simulink model "EV_Truck_Model"  (R2022b)
settings: Solver=FixedStepAuto  StartTime=0  StopTime=26553  FixedStep=0.1  RelTol=1e-3
model workspace (MAT data in the model file):
  ADAS_MaxAccel = 2
  ADAS_MaxDecel = 2.5
  Adas_on_off = 0
  Batt_cap_ah : Simulink.Parameter (value not decoded)
  Batt_rist_r0 : Simulink.Parameter (value not decoded)
  Batt_soc_s0 : Simulink.Parameter (value not decoded)
  Batt_volt_v0 : Simulink.Parameter (value not decoded)
  Motor_eff_100 : Simulink.Parameter (value not decoded)
  Motor_eff_190 : Simulink.Parameter (value not decoded)
  Motor_eff_95 : Simulink.Parameter (value not decoded)
  Motor_rpm_100 : Simulink.Parameter (value not decoded)
  Motor_rpm_190 : Simulink.Parameter (value not decoded)
  Motor_rpm_95 : Simulink.Parameter (value not decoded)
  Motor_torque_pos_100 : Simulink.Parameter (value not decoded)
  Motor_torque_pos_190 : Simulink.Parameter (value not decoded)
  Motor_torque_pos_95 : Simulink.Parameter (value not decoded)
  Motor_trq_190 : Simulink.Parameter (value not decoded)
  Motor_trq_95 : Simulink.Parameter (value not decoded)
  Sim_step = 0.1
  Test_DriveCycle = 0
  Trans_ratio = 6.142
  Veh_cog_fx = 1.69543
  Veh_cog_h = 0.605887
  Veh_cog_rx = 2.11956
  Veh_diff = 6.7
  Veh_whl_crr = 0.01
  Veh_whl_k = 180000
  Veh_whl_radius = 0.35
symbols that are objects in the model workspace (value not decoded): Motor_eff_100, Motor_eff_190, Motor_eff_95, Motor_rpm_100, Motor_rpm_190, Motor_rpm_95, Motor_torque_pos_100, Motor_torque_pos_190, Motor_torque_pos_95, Motor_trq_190, Motor_trq_95
undefined symbols (not defined in the file): Batt_soc_init, canChannel, Elec_aux_sw, Elec_rgn_sw, Power_option, speed, time, Veh_mass
libraries: batteryecm_lib x170, simulink x14, canmsglib x9, canlib x7, autolibshared x5, nesl_utility x4, fl_lib x3, drivingvehiclecontroller x3, hdlsllib x3, sim3dlib x1, sim3dautolib x1, vrlib x1
(part 11 of 11)

== stateflow chart EV_Truck_Model/VCU/Remap Subsystem/VCU_TorqueCommand ==
  state CruiseControl [commented out]
    state TooSlow [commented out]
      TrqCmd = TrqCmd + 5* ...
      abs(Speed-ADAS_speed);
      state NoBrake [commented out]
      state Brake [commented out]
        BrakeCmd = ...
        BrakeCmd + 5;
      (default) -> NoBrake [commented out]
      NoBrake -> CruiseControl.TooSlow.Brake [commented out] : [TrqCmd<0]
    state InitialState [commented out]
      TrqCmd = 100;
    state TooFast [commented out]
      TrqCmd = TrqCmd - 5* ...
      abs(Speed-ADAS_speed);
      BrakeCmd = 0;
    state PerfectCondition [commented out]
      %No Command
    state Error [commented out]
      ADAS_fault = 1;
    state TempState [commented out]
      %Wait 0.1 sec
    (default) -> InitialState [commented out]
    InitialState -> PerfectCondition [commented out]
    (junction 250) -> TooFast [commented out] : [Speed > ADAS_speed+2.0]
    (junction 250) -> TooSlow [commented out] : [Speed < ADAS_speed-2.0]
    (junction 250) -> Error [commented out] : [abs(Speed-ADAS_speed)>10]
    TooFast -> TempState [commented out]
    PerfectCondition -> (junction 250) [commented out]
    TempState -> PerfectCondition [commented out] : after(0.1,sec)
    TooSlow -> TempState [commented out]
  state AdaptiveCruiseControl [commented out]
    TargetDistance = Speed*(1+(ADAS_mode-3)*0.1)/2+1;
    if 1/TTC < 0.1
    ADAS_SpdCmd = ADAS_speed;
    else
    ADAS_SpdCmd = ADAS_speed;
    end
  state Initialize
    state BOTS [parallel]
      settings: executionOrder=1
      state BrakeFactor0
        BrakeFactor=0;
      state BrakeFactor1
        BrakeFactor=1;
      Initialize.BOTS.BrakeFactor0 -> Initialize.BOTS.BrakeFactor1 : [Brake > 0]
      (default) -> Initialize.BOTS.BrakeFactor1
      Initialize.BOTS.BrakeFactor1 -> Initialize.BOTS.BrakeFactor0 : [Brake == 0]
    state RegenTriggerCriteria [parallel]
      settings: executionOrder=2
      state RegenOff
        Regen = 0;
        DCRegen = 0;
      state RegenOn
        Regen = 1;
        DCRegen = 1;
      RegenOff -> RegenOn : [RPM>200&&(RegenSW==1||DCRegenSW==1)&&SOC<=0.95]
      (default) -> RegenOff
      RegenOn -> RegenOff : [RPM<200||(RegenSW==0&&DCRegenSW==0)||SOC>0.95]
    state DriveCycleTset [parallel] [commented out]
    state ADASTriggerCriteria [parallel]
      settings: executionOrder=3
      state CruiseOff
        ADAS = 0;
        ADAS_fault = 0;
      state CruiseOn
        ADAS = 1;
        state PLUSTEMP
          %Stop increase
        state PLUS
          ADAS_speed...
          =ADAS_speed+1;
        state PLUSTEMP5
          %Stop increase
        state PLUS5
          ADAS_speed...
          =ADAS_speed+5;
        state IC
          ADAS_speed = ...
          Speed;
          %1 Time Only
        state NC
          %No Command
        state MINUSTEMP
          %Stop decrease
        state MINUS
          ADAS_speed...
          =ADAS_speed-1;
        state MINUSTEMP5
          %Stop decrease
        state MINUS5
          ADAS_speed...
          =ADAS_speed-5;
        PLUSTEMP -> PLUS5 [order 2] : after(0.75,sec)
        PLUS5 -> PLUSTEMP5
        NC -> PLUSTEMP [order 1] : [ADAS_add == 1]
        PLUSTEMP5 -> (junction 376) [order 2] : [ADAS_add == 0]
        PLUS -> (junction 215)
        PLUSTEMP -> PLUS [order 1] : [ADAS_add == 0]
        PLUSTEMP5 -> PLUS5 [order 1] : after(0.25,sec)
        (default) -> IC
        (junction 376) -> (junction 215)
        (junction 215) -> NC
        MINUSTEMP5 -> (junction 376) [order 2] : [ADAS_min == 0]
        MINUS -> (junction 215)
        IC -> NC
        MINUS5 -> MINUSTEMP5
        MINUSTEMP -> MINUS [order 2] : [ADAS_min == 0]
        NC -> MINUSTEMP [order 2] : [ADAS_min == 1]
        MINUSTEMP -> MINUS5 [order 1] : after(0.75,sec)
        MINUSTEMP5 -> MINUS5 [order 1] : after(0.25,sec)
      state CruiseReady
        ADAS = 0;
        ADAS_speed ...
        =0;
      state CruiseTest
        ADAS = 1;
        ADAS_speed=ADAS_speed_profile;
      CruiseReady -> CruiseOff [order 2] : [ADAS_on == 0]
      (default) -> CruiseOff
      CruiseOn -> CruiseReady : [ADAS_enable == 0 || ADAS_on == 0 || ADAS_fault == 1 || BrakeFactor ==1]
      CruiseOff -> CruiseReady : [ADAS_on == 1]
      CruiseReady -> CruiseTest [order 3] : [ADAS_test == 1]
      CruiseReady -> CruiseOn [order 1] : [ADAS_enable == 1 && BrakeFactor== 0 && Speed > 20]
    state ThrottleMapping [parallel]
      settings: executionOrder=4
      state Initiation
        ADAS_SpdCmd = 0;
        state CruiseControl
          state TrqCmdMapping [parallel]
            settings: executionOrder=1
            state NoRegen
              TrqCmd = ADAS_AccelCmd ...
              /2*600;
              BrakeCmd = ADAS_DecelCmd ...
              /2.5*600;
            state Regen
              TrqCmd = ADAS_AccelCmd ...
              /2*600;
              BrakeCmd = ADAS_DecelCmd ...
              /2.5*600;
            state AdaptiveCruiseControlException
              TrqCmd = 0;
            Regen -> NoRegen [order 1] : [Regen == 0]
            NoRegen -> Regen [order 1] : [Regen == 1]
            NoRegen -> (junction 412) [order 2]
            Regen -> (junction 412) [order 2]
            (junction 412) -> AdaptiveCruiseControlException : [ADAS_exception == 1]
            AdaptiveCruiseControlException -> NoRegen : [ADAS_exception == 0]
          state ControlState [parallel]
            ADAS_activate = 1;
            settings: executionOrder=2
            state CruiseControl
              ADAS_SpdCmd = ADAS_speed;
              state ErrorState
                ADAS_fault = 1;
                ADAS_activate = 0;
              state ErrorCheck
              ErrorCheck -> ErrorState : [abs(Speed-ADAS_speed)>10 && after(1,sec)&&ADAS_test==0]
              (default) -> ErrorCheck
            state AdaptiveCruiseControl
              TargetDistance = Speed* ...
              (1+(ADAS_mode-3)*0.1)/2+0.5;
              if ADAS_SpdCmd > ADAS_speed
              ADAS_SpdCmd = ADAS_speed;
              end
              state Brake
                ADAS_exception =1;
                ADAS_SpdCmd = 5;
                state CrashDanger
                  BrakeCmd = 1000;
                state ApplyBrake
                  BrakeCmd = 500/TTC;
                ApplyBrake -> CrashDanger : [TTC<0.5]
                CrashDanger -> ApplyBrake : [TTC>=0.5]
                (default) -> ApplyBrake
              state StillFarAway
                ADAS_SpdCmd = ADAS_speed;
                if ADAS_Speed_Deltakph < -10
                ADAS_SpdCmd = Speed+ ...
                ADAS_Speed_Deltakph/ ...
                (ADAS_Distance- ...
                TargetDistance);
                elseif ADAS_Speed_Deltakph > 5
                ADAS_SpdCmd = Speed+ ...
                ADAS_Speed_Deltakph;
                end
                if ADAS_SpdCmd > ADAS_speed
                ADAS_SpdCmd = ADAS_speed;
                end
              state TooFarAway
                ADAS_SpdCmd ...
                = ADAS_speed;
              state MaintainDistance
                ADAS_SpdCmd = Speed+ ...
                ADAS_Speed_Deltakph;
                ADAS_exception =0;
                if ADAS_SpdCmd > ADAS_speed
                ADAS_SpdCmd = ADAS_speed;
                end
              Initialize.ThrottleMapping.Initiation.CruiseControl.ControlState.AdaptiveCruiseControl.Brake -> MaintainDistance : [TTC>=5]
              MaintainDistance -> Initialize.ThrottleMapping.Initiation.CruiseControl.ControlState.AdaptiveCruiseControl.Brake [order 2] : [TTC<5]
              (default) -> TooFarAway
              StillFarAway -> TooFarAway [order 2] : [ADAS_Distance >= 200]
              TooFarAway -> StillFarAway : [ADAS_Distance < 200]
              MaintainDistance -> StillFarAway [order 1] : [ADAS_Distance >= TargetDistance]
              StillFarAway -> MaintainDistance [order 1] : [ADAS_Distance < TargetDistance]
            (default) -> Initialize.ThrottleMapping.Initiation.CruiseControl.ControlState.CruiseControl
            Initialize.ThrottleMapping.Initiation.CruiseControl.ControlState.CruiseControl -> Initialize.ThrottleMapping.Initiation.CruiseControl.ControlState.AdaptiveCruiseControl : [ADAS_mode ~= 0]
            Initialize.ThrottleMapping.Initiation.CruiseControl.ControlState.AdaptiveCruiseControl -> Initialize.ThrottleMapping.Initiation.CruiseControl.ControlState.CruiseControl : [ADAS_mode == 0]
          (default) -> NoRegen
        state ForwardGear
          ADAS_activate = 0;
          state OPD
            state TrqCmd_Regen
              state TrqCmd_Positive
                TrqCmd = TrqLimit_Pos* ...
                (Throttle-40)/160;
                BrakeCmd = 0;
              state TrqCmd_Negative
                TrqCmd = ...
                -100+100 ...
                *Throttle/40;
                BrakeCmd = 0;
              state Brake
                state Brake_RGN
                  TrqCmd = -100 ...
                  -200*Brake/150;
                  BrakeCmd = 450 ...
                  *Brake/150;
                state Brake_NoTrq
                  TrqCmd = 0;
                  BrakeCmd = ...
                  Brake*5;
                (default) -> Initialize.ThrottleMapping.Initiation.ForwardGear.OPD.TrqCmd_Regen.Brake.Brake_RGN
                Initialize.ThrottleMapping.Initiation.ForwardGear.OPD.TrqCmd_Regen.Brake.Brake_NoTrq -> Initialize.ThrottleMapping.Initiation.ForwardGear.OPD.TrqCmd_Regen.Brake.Brake_RGN : [Brake < 150]
                Initialize.ThrottleMapping.Initiation.ForwardGear.OPD.TrqCmd_Regen.Brake.Brake_RGN -> Initialize.ThrottleMapping.Initiation.ForwardGear.OPD.TrqCmd_Regen.Brake.Brake_NoTrq : [Brake > 150]
              (default) -> Initialize.ThrottleMapping.Initiation.ForwardGear.OPD.TrqCmd_Regen.TrqCmd_Positive
              Initialize.ThrottleMapping.Initiation.ForwardGear.OPD.TrqCmd_Regen.TrqCmd_Negative -> Initialize.ThrottleMapping.Initiation.ForwardGear.OPD.TrqCmd_Regen.TrqCmd_Positive [order 2] : [Throttle >= 40]
              Initialize.ThrottleMapping.Initiation.ForwardGear.OPD.TrqCmd_Regen.TrqCmd_Positive -> Initialize.ThrottleMapping.Initiation.ForwardGear.OPD.TrqCmd_Regen.TrqCmd_Negative [order 1] : [Throttle < 40]
              Initialize.ThrottleMapping.Initiation.ForwardGear.OPD.TrqCmd_Regen.TrqCmd_Positive -> (junction 74) [order 2]
              Initialize.ThrottleMapping.Initiation.ForwardGear.OPD.TrqCmd_Regen.TrqCmd_Negative -> (junction 74) [order 1]
              (junction 74) -> Initialize.ThrottleMapping.Initiation.ForwardGear.OPD.TrqCmd_Regen.Brake : [BrakeFactor ==1]
              Initialize.ThrottleMapping.Initiation.ForwardGear.OPD.TrqCmd_Regen.Brake -> Initialize.ThrottleMapping.Initiation.ForwardGear.OPD.TrqCmd_Regen.TrqCmd_Negative : [BrakeFactor == 0]
            state NoTrqCmd
              TrqCmd = 0;
              BrakeCmd = ...
              Brake*5;
            state TrqCmd_Normal
              TrqCmd = ...
              TrqLimit_Pos*...
              Throttle/200;
              BrakeCmd = 0;
            (default) -> Initialize.ThrottleMapping.Initiation.ForwardGear.OPD.NoTrqCmd
            Initialize.ThrottleMapping.Initiation.ForwardGear.OPD.TrqCmd_Normal -> Initialize.ThrottleMapping.Initiation.ForwardGear.OPD.NoTrqCmd [order 2] : [BrakeFactor == 1]
            Initialize.ThrottleMapping.Initiation.ForwardGear.OPD.NoTrqCmd -> Initialize.ThrottleMapping.Initiation.ForwardGear.OPD.TrqCmd_Normal : [BrakeFactor == 0]
            Initialize.ThrottleMapping.Initiation.ForwardGear.OPD.TrqCmd_Regen -> Initialize.ThrottleMapping.Initiation.ForwardGear.OPD.TrqCmd_Normal : [Regen == 0]
            Initialize.ThrottleMapping.Initiation.ForwardGear.OPD.TrqCmd_Normal -> Initialize.ThrottleMapping.Initiation.ForwardGear.OPD.TrqCmd_Regen [order 1] : [Regen == 1]
          state non_OPD
            state TrqCmd_Regen
              state TrqCmd
                TrqCmd = TrqLimit_Pos* ...
                Throttle/200;
                BrakeCmd = 0;
              state Brake
                state Brake_RGN
                  TrqCmd = -300* ...
                  Brake/150;
                  BrakeCmd = 450 ...
                  *Brake/150;
                state Brake_NoTrq
                  TrqCmd = 0;
                  BrakeCmd = ...
                  Brake*5;
                (default) -> Initialize.ThrottleMapping.Initiation.ForwardGear.non_OPD.TrqCmd_Regen.Brake.Brake_RGN
                Initialize.ThrottleMapping.Initiation.ForwardGear.non_OPD.TrqCmd_Regen.Brake.Brake_NoTrq -> Initialize.ThrottleMapping.Initiation.ForwardGear.non_OPD.TrqCmd_Regen.Brake.Brake_RGN : [Brake < 150]
                Initialize.ThrottleMapping.Initiation.ForwardGear.non_OPD.TrqCmd_Regen.Brake.Brake_RGN -> Initialize.ThrottleMapping.Initiation.ForwardGear.non_OPD.TrqCmd_Regen.Brake.Brake_NoTrq : [Brake > 150]
              (default) -> Initialize.ThrottleMapping.Initiation.ForwardGear.non_OPD.TrqCmd_Regen.TrqCmd
              Initialize.ThrottleMapping.Initiation.ForwardGear.non_OPD.TrqCmd_Regen.Brake -> Initialize.ThrottleMapping.Initiation.ForwardGear.non_OPD.TrqCmd_Regen.TrqCmd : [BrakeFactor == 0]
              Initialize.ThrottleMapping.Initiation.ForwardGear.non_OPD.TrqCmd_Regen.TrqCmd -> Initialize.ThrottleMapping.Initiation.ForwardGear.non_OPD.TrqCmd_Regen.Brake : [BrakeFactor == 1]
            state NoTrqCmd
              TrqCmd = 0;
              BrakeCmd = ...
              Brake*5;
            state TrqCmd_Normal
              TrqCmd = ...
              TrqLimit_Pos*...
              Throttle/200;
              BrakeCmd = 0;
            (default) -> Initialize.ThrottleMapping.Initiation.ForwardGear.non_OPD.NoTrqCmd
            Initialize.ThrottleMapping.Initiation.ForwardGear.non_OPD.TrqCmd_Normal -> Initialize.ThrottleMapping.Initiation.ForwardGear.non_OPD.NoTrqCmd [order 2] : [BrakeFactor == 1]
            Initialize.ThrottleMapping.Initiation.ForwardGear.non_OPD.NoTrqCmd -> Initialize.ThrottleMapping.Initiation.ForwardGear.non_OPD.TrqCmd_Normal : [BrakeFactor == 0]
            Initialize.ThrottleMapping.Initiation.ForwardGear.non_OPD.TrqCmd_Regen -> Initialize.ThrottleMapping.Initiation.ForwardGear.non_OPD.TrqCmd_Normal : [Regen == 0]
            Initialize.ThrottleMapping.Initiation.ForwardGear.non_OPD.TrqCmd_Normal -> Initialize.ThrottleMapping.Initiation.ForwardGear.non_OPD.TrqCmd_Regen [order 1] : [Regen == 1]
          Initialize.ThrottleMapping.Initiation.ForwardGear.OPD -> Initialize.ThrottleMapping.Initiation.ForwardGear.non_OPD : [OPDSW == 0]
          Initialize.ThrottleMapping.Initiation.ForwardGear.non_OPD -> Initialize.ThrottleMapping.Initiation.ForwardGear.OPD : [OPDSW == 1]
          (default) -> Initialize.ThrottleMapping.Initiation.ForwardGear.non_OPD
        state NeutralGear
          TrqCmd = 0;
          BrakeCmd = Brake*5;
        state ReverseGear
          TrqCmd = Throttle/200* ...
          TrqLimit_Neg*0.75;
          BrakeCmd = Brake*5;
        (default) -> Initialize.ThrottleMapping.Initiation.NeutralGear
        (junction 319) -> Initialize.ThrottleMapping.Initiation.NeutralGear : [Gear == 0]
        Initialize.ThrottleMapping.Initiation.NeutralGear -> (junction 317) [order 2]
        Initialize.ThrottleMapping.Initiation.NeutralGear -> (junction 315) [order 1]
        Initialize.ThrottleMapping.Initiation.ForwardGear -> (junction 319) [order 2]
        Initialize.ThrottleMapping.Initiation.ReverseGear -> (junction 319) [order 2]
        (junction 315) -> Initialize.ThrottleMapping.Initiation.ForwardGear : [Gear ==1]
        Initialize.ThrottleMapping.Initiation.ReverseGear -> (junction 315) [order 1]
        Initialize.ThrottleMapping.Initiation.ForwardGear -> (junction 317) [order 3]
        (junction 317) -> Initialize.ThrottleMapping.Initiation.ReverseGear : [Gear == 2]
        Initialize.ThrottleMapping.Initiation.ForwardGear -> Initialize.ThrottleMapping.Initiation.CruiseControl [order 1] : [ADAS == 1]
        Initialize.ThrottleMapping.Initiation.CruiseControl -> Initialize.ThrottleMapping.Initiation.ForwardGear : [ADAS == 0]
      state DriveCycleTest
        ADAS_SpdCmd = 0;
        note: Throttle Command 0-200
            | Brake Command 0-200
            | 4 State:
            | OPD on/off
            | RGN on/off
        state TorqueCommand [parallel]
          settings: executionOrder=1
          state ForwardGear
            ADAS_activate = 0;
            state OPD [commented out]
              state TrqCmd_Regen [commented out]
                state TrqCmd_Positive [commented out]
                  TrqCmd = TrqLimit_Pos* ...
                  (DCThrottle-40)/160;
                  BrakeCmd = 0;
                state TrqCmd_Negative [commented out]
                  TrqCmd = ...
                  -100+100 ...
                  *DCThrottle/40;
                  BrakeCmd = 0;
                state Brake [commented out]
                  state Brake_RGN [commented out]
                    TrqCmd = -100 ...
                    -200*DCBrake/150;
                    BrakeCmd = 450 ...
                    *DCBrake/150;
                  state Brake_NoTrq [commented out]
                    TrqCmd = 0;
                    BrakeCmd = ...
                    DCBrake*5;
                  (default) -> Initialize.ThrottleMapping.DriveCycleTest.TorqueCommand.ForwardGear.OPD.TrqCmd_Regen.Brake.Brake_RGN [commented out]
                  Initialize.ThrottleMapping.DriveCycleTest.TorqueCommand.ForwardGear.OPD.TrqCmd_Regen.Brake.Brake_NoTrq -> Initialize.ThrottleMapping.DriveCycleTest.TorqueCommand.ForwardGear.OPD.TrqCmd_Regen.Brake.Brake_RGN [commented out] : [DCBrake < 150]
                  Initialize.ThrottleMapping.DriveCycleTest.TorqueCommand.ForwardGear.OPD.TrqCmd_Regen.Brake.Brake_RGN -> Initialize.ThrottleMapping.DriveCycleTest.TorqueCommand.ForwardGear.OPD.TrqCmd_Regen.Brake.Brake_NoTrq [commented out] : [DCBrake > 150]
                (default) -> Initialize.ThrottleMapping.DriveCycleTest.TorqueCommand.ForwardGear.OPD.TrqCmd_Regen.TrqCmd_Positive [commented out]
                Initialize.ThrottleMapping.DriveCycleTest.TorqueCommand.ForwardGear.OPD.TrqCmd_Regen.TrqCmd_Negative -> Initialize.ThrottleMapping.DriveCycleTest.TorqueCommand.ForwardGear.OPD.TrqCmd_Regen.TrqCmd_Positive [commented out] : [DCThrottle >= 40]
                Initialize.ThrottleMapping.DriveCycleTest.TorqueCommand.ForwardGear.OPD.TrqCmd_Regen.TrqCmd_Positive -> Initialize.ThrottleMapping.DriveCycleTest.TorqueCommand.ForwardGear.OPD.TrqCmd_Regen.TrqCmd_Negative [commented out] : [DCThrottle < 40]
                Initialize.ThrottleMapping.DriveCycleTest.TorqueCommand.ForwardGear.OPD.TrqCmd_Regen.TrqCmd_Positive -> (junction 435) [commented out]
                Initialize.ThrottleMapping.DriveCycleTest.TorqueCommand.ForwardGear.OPD.TrqCmd_Regen.TrqCmd_Negative -> (junction 435) [commented out]
                (junction 435) -> Initialize.ThrottleMapping.DriveCycleTest.TorqueCommand.ForwardGear.OPD.TrqCmd_Regen.Brake [commented out] : [DCBrakeFactor ==1]
                Initialize.ThrottleMapping.DriveCycleTest.TorqueCommand.ForwardGear.OPD.TrqCmd_Regen.Brake -> Initialize.ThrottleMapping.DriveCycleTest.TorqueCommand.ForwardGear.OPD.TrqCmd_Regen.TrqCmd_Negative [commented out] : [DCBrakeFactor == 0]
              state NoTrqCmd [commented out]
                TrqCmd = 0;
                BrakeCmd = ...
                DCBrake*5;
              state TrqCmd_Normal [commented out]
                TrqCmd = ...
                TrqLimit_Pos*...
                DCThrottle/200;
                BrakeCmd = 0;
              (default) -> Initialize.ThrottleMapping.DriveCycleTest.TorqueCommand.ForwardGear.OPD.NoTrqCmd [commented out]
              Initialize.ThrottleMapping.DriveCycleTest.TorqueCommand.ForwardGear.OPD.TrqCmd_Normal -> Initialize.ThrottleMapping.DriveCycleTest.TorqueCommand.ForwardGear.OPD.NoTrqCmd [commented out] : [BrakeFactor == 1]
              Initialize.ThrottleMapping.DriveCycleTest.TorqueCommand.ForwardGear.OPD.NoTrqCmd -> Initialize.ThrottleMapping.DriveCycleTest.TorqueCommand.ForwardGear.OPD.TrqCmd_Normal [commented out] : [BrakeFactor == 0]
              Initialize.ThrottleMapping.DriveCycleTest.TorqueCommand.ForwardGear.OPD.TrqCmd_Regen -> Initialize.ThrottleMapping.DriveCycleTest.TorqueCommand.ForwardGear.OPD.TrqCmd_Normal [commented out] : [Regen == 0]
              Initialize.ThrottleMapping.DriveCycleTest.TorqueCommand.ForwardGear.OPD.TrqCmd_Normal -> Initialize.ThrottleMapping.DriveCycleTest.TorqueCommand.ForwardGear.OPD.TrqCmd_Regen [commented out] : [Regen == 1]
            state non_OPD
              state TrqCmd_Regen
                state TrqCmd
                  TrqCmd = TrqLimit_Pos* ...
                  DCThrottle/200;
                  BrakeCmd = 0;
                state Brake
                  state Brake_RGN
                    TrqCmd = -300* ...
                    DCBrake/150;
                    BrakeCmd = 450 ...
                    *DCBrake/150;
                  state Brake_NoTrq
                    TrqCmd = 0;
                    BrakeCmd = ...
                    DCBrake*5;
                  (default) -> Initialize.ThrottleMapping.DriveCycleTest.TorqueCommand.ForwardGear.non_OPD.TrqCmd_Regen.Brake.Brake_RGN
                  Initialize.ThrottleMapping.DriveCycleTest.TorqueCommand.ForwardGear.non_OPD.TrqCmd_Regen.Brake.Brake_NoTrq -> Initialize.ThrottleMapping.DriveCycleTest.TorqueCommand.ForwardGear.non_OPD.TrqCmd_Regen.Brake.Brake_RGN : [DCBrake < 150]
                  Initialize.ThrottleMapping.DriveCycleTest.TorqueCommand.ForwardGear.non_OPD.TrqCmd_Regen.Brake.Brake_RGN -> Initialize.ThrottleMapping.DriveCycleTest.TorqueCommand.ForwardGear.non_OPD.TrqCmd_Regen.Brake.Brake_NoTrq : [DCBrake > 150]
                (default) -> Initialize.ThrottleMapping.DriveCycleTest.TorqueCommand.ForwardGear.non_OPD.TrqCmd_Regen.TrqCmd
                Initialize.ThrottleMapping.DriveCycleTest.TorqueCommand.ForwardGear.non_OPD.TrqCmd_Regen.Brake -> Initialize.ThrottleMapping.DriveCycleTest.TorqueCommand.ForwardGear.non_OPD.TrqCmd_Regen.TrqCmd : [DCBrakeFactor == 0]
                Initialize.ThrottleMapping.DriveCycleTest.TorqueCommand.ForwardGear.non_OPD.TrqCmd_Regen.TrqCmd -> Initialize.ThrottleMapping.DriveCycleTest.TorqueCommand.ForwardGear.non_OPD.TrqCmd_Regen.Brake : [DCBrakeFactor == 1]
              state NoTrqCmd
                TrqCmd = 0;
                BrakeCmd = ...
                DCBrake*5;
              state TrqCmd_Normal
                TrqCmd = ...
                TrqLimit_Pos*...
                DCThrottle/200;
                BrakeCmd = 0;
              (default) -> Initialize.ThrottleMapping.DriveCycleTest.TorqueCommand.ForwardGear.non_OPD.NoTrqCmd
              Initialize.ThrottleMapping.DriveCycleTest.TorqueCommand.ForwardGear.non_OPD.TrqCmd_Normal -> Initialize.ThrottleMapping.DriveCycleTest.TorqueCommand.ForwardGear.non_OPD.NoTrqCmd [order 1] : [DCBrakeFactor == 1]
              Initialize.ThrottleMapping.DriveCycleTest.TorqueCommand.ForwardGear.non_OPD.NoTrqCmd -> Initialize.ThrottleMapping.DriveCycleTest.TorqueCommand.ForwardGear.non_OPD.TrqCmd_Normal : [DCBrakeFactor == 0]
              Initialize.ThrottleMapping.DriveCycleTest.TorqueCommand.ForwardGear.non_OPD.TrqCmd_Regen -> Initialize.ThrottleMapping.DriveCycleTest.TorqueCommand.ForwardGear.non_OPD.TrqCmd_Normal : [DCRegen == 0]
              Initialize.ThrottleMapping.DriveCycleTest.TorqueCommand.ForwardGear.non_OPD.TrqCmd_Normal -> Initialize.ThrottleMapping.DriveCycleTest.TorqueCommand.ForwardGear.non_OPD.TrqCmd_Regen [order 2] : [DCRegen == 1]
            Initialize.ThrottleMapping.DriveCycleTest.TorqueCommand.ForwardGear.OPD -> Initialize.ThrottleMapping.DriveCycleTest.TorqueCommand.ForwardGear.non_OPD [commented out] : [OPDSW == 0]
            Initialize.ThrottleMapping.DriveCycleTest.TorqueCommand.ForwardGear.non_OPD -> Initialize.ThrottleMapping.DriveCycleTest.TorqueCommand.ForwardGear.OPD [commented out] : [OPDSW == 1]
            (default) -> Initialize.ThrottleMapping.DriveCycleTest.TorqueCommand.ForwardGear.non_OPD
          state NeutralGear
            TrqCmd = 0;
            BrakeCmd = DCBrake*5;
          state ReverseGear
            TrqCmd = DCThrottle/200* ...
            TrqLimit_Neg*0.75;
            BrakeCmd = DCBrake*5;
          (default) -> Initialize.ThrottleMapping.DriveCycleTest.TorqueCommand.NeutralGear
          (junction 488) -> Initialize.ThrottleMapping.DriveCycleTest.TorqueCommand.NeutralGear : [Gear == 0]
          Initialize.ThrottleMapping.DriveCycleTest.TorqueCommand.NeutralGear -> (junction 463) [order 2]
          Initialize.ThrottleMapping.DriveCycleTest.TorqueCommand.NeutralGear -> (junction 471) [order 1]
          Initialize.ThrottleMapping.DriveCycleTest.TorqueCommand.ForwardGear -> (junction 488) [order 1]
          Initialize.ThrottleMapping.DriveCycleTest.TorqueCommand.ReverseGear -> (junction 488) [order 2]
          (junction 471) -> Initialize.ThrottleMapping.DriveCycleTest.TorqueCommand.ForwardGear : [Gear ==1]
          Initialize.ThrottleMapping.DriveCycleTest.TorqueCommand.ReverseGear -> (junction 471) [order 1]
          Initialize.ThrottleMapping.DriveCycleTest.TorqueCommand.ForwardGear -> (junction 463) [order 2]
          (junction 463) -> Initialize.ThrottleMapping.DriveCycleTest.TorqueCommand.ReverseGear : [Gear == 2]
        state TorqueMapping [parallel]
          settings: executionOrder=2
          state AccelCmd
            DCThrottle = (DriveCycleAccelCmd/3)*200;
            %1000Nm = 3.3m/s^2 acceleration
            %Throttle 200 = 1000Nm
            DCBrake = 0;
          state DecelCmd
            DCThrottle = 0;
            DCBrake = DriveCycleDecelCmd/3.5*200;
          (default) -> AccelCmd
          AccelCmd -> DecelCmd : [DriveCycleDecelCmd>0]
          DecelCmd -> AccelCmd : [DriveCycleAccelCmd>0]
        state BOTS [parallel]
          settings: executionOrder=3
          state BrakeFactor0
            DCBrakeFactor=0;
          state BrakeFactor1
            DCBrakeFactor=1;
          Initialize.ThrottleMapping.DriveCycleTest.BOTS.BrakeFactor0 -> Initialize.ThrottleMapping.DriveCycleTest.BOTS.BrakeFactor1 : [DCBrake > 0]
          (default) -> Initialize.ThrottleMapping.DriveCycleTest.BOTS.BrakeFactor1
          Initialize.ThrottleMapping.DriveCycleTest.BOTS.BrakeFactor1 -> Initialize.ThrottleMapping.DriveCycleTest.BOTS.BrakeFactor0 : [DCBrake == 0]
      (default) -> Initiation
      DriveCycleTest -> Initiation : [DriveCycleEnable == 0]
      Initiation -> DriveCycleTest : [DriveCycleEnable == 1]
  data: ADAS_AccelCmd input; ADAS_DecelCmd input; DriveCycleEnable input; DriveCycleAccelCmd input; DriveCycleDecelCmd input; ADAS_on input; ADAS_enable input; ADAS_add input; ADAS_min input; ADAS_Speed_Delta input; ADAS_Speed_Deltakph input; ADAS_mode input; Speed input; TTC input; TrqLimit_Pos input; TrqLimit_Neg input; RPM input; Throttle input; Brake input; OPDSW input; RegenSW input; TrqCmd output [-1000..1000] =0; BrakeFactor local =0; SOC input; BrakeCmd output [0..1000] =0; ADAS local =0; ADAS_speed local double =0; Gear input; ADAS_activate output =0; ADAS_fault output =0; TargetDistance local =0; ADAS_Distance input; Regen output =0; ADAS_SpdCmd output =0; ADAS_exception local =0; DCBrake local =0; DCBrakeFactor local =0; DCThrottle local =0; DCRegenSW input; DCRegen local; ADAS_speed_profile input; ADAS_test input

== stateflow chart EV_Truck_Model/Vehicle Dynamics System/Power Delivery and Braking System/GearBox/Chart ==

== stateflow chart EV_Truck_Model/System I//O/Control Mode/Counter ==
  state Initial
    count = 0;
  state add
    count = count+1;
  state add1
    count = count-1;
  (default) -> Initial
  Initial -> add
  add -> add1 : [count == 15]
  add1 -> add : [count == 0]
  data: count output
